simulink model "sschdlexSwissRectifierModel"  (R2026a)
settings: Solver=FixedStepDiscrete  StopTime=.03  AbsTol=1e-3
PostLoadFcn:
  | SolverConfiguration1_Gs = Simulink.Parameter;
  | SolverConfiguration1_Gs.Value = 1;
  | SolverConfiguration1_s = Simulink.Parameter;
  | SolverConfiguration1_s.Value = 1;
InitFcn:
  | freqMain = 50;
  | Vrms=230;
  | Vin = Vrms * sqrt(2);
  | Vout=325;
  | freqSwitch=20e3;
  | PoutMax = 7.5e3;
  | loadPercent = 50;
  | RLoad = Vout^2/(PoutMax*(loadPercent/100));
  | COut = 470e-6;
  | LDC = 305e-6;
  | LF = 85e-6;
  | CF = 4.4e-6;
undefined symbols (not defined in the file or in its folder): Down, Up
libraries: fl_lib x36, SimscapeFPGAHIL_lib x22, nesl_utility x9, simulink x2, slpidlib x2, eeGeneralControl x1
settings Model: DataTypeOverride=Off  Creator=The MathWorks, Inc.  LastModifiedBy=The MathWorks, Inc.
settings OptimizationCC: ConditionallyExecuteInputs=off
settings DebuggingCC: AlgebraicLoopMsg=error  SingleTaskRateTransMsg=error  PregeneratedLibrarySubsystemCodeDiagnostic=none
settings HardwareCC: ProdHWDeviceType=ASIC/FPGA->ASIC/FPGA  TargetBitPerLong=64.0  TargetBitPerPointer=64.0  TargetBitPerSizeT=64.0  TargetBitPerPtrDiffT=64.0  TargetLongLongMode=on  TargetIntDivRoundTo=Zero  TargetEndianess=LittleEndian  TargetWordSize=64.0  TargetHWDeviceType=Custom Processor->MATLAB Host Computer  ProdEqTarget=off
settings SimscapeCC: SimscapeNominalValues="[{\"value\":\"1\",\"unit\":\"A\"},{\"value\":\"1\",\"unit\":\"bar\"},{\"value\":\"1\",\"unit\":\"cm^2\"},{\"value\":\"1\",\"unit\":\"cm^3/s\"},{\"value\":\"1\",\"unit\":\"kJ/kg\"},{\"value\":\"1\",\"unit\":\"kW\"},{\"value\":\"1\",\"unit\":\"l\"},{\"value\":\"1\",\"unit\":\"N\"},{\"value\":\"1\",\"unit\":\"N*m\"},{\"value\":\"1\",\"unit\":\"V\"}]"

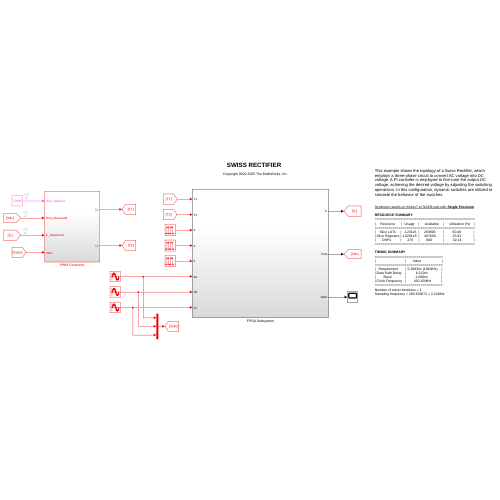
[thumbnail: Simulink's stored preview of the top-level diagram]
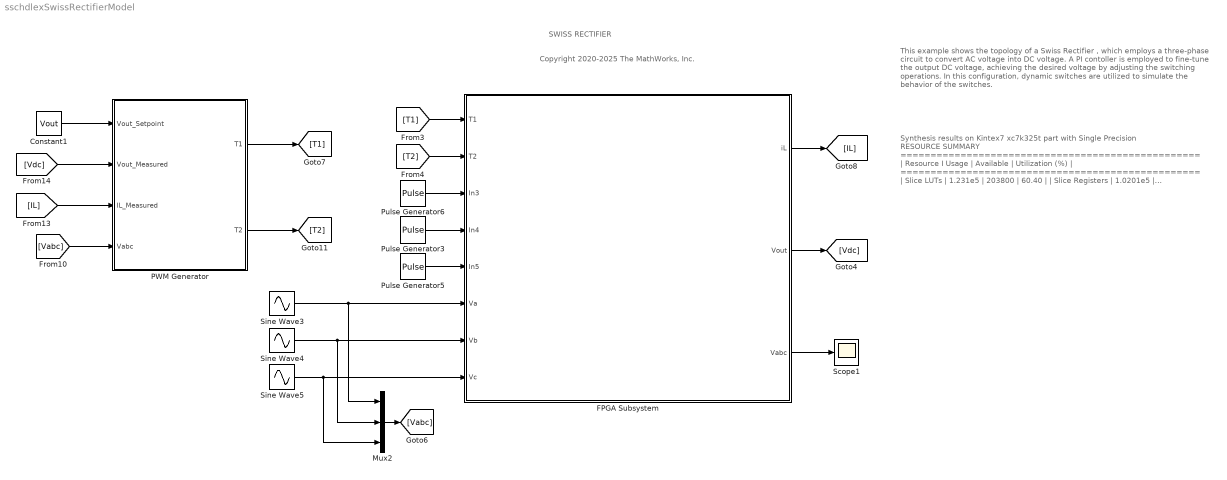
== system sschdlexSwissRectifierModel ==
  note: SWISS RECTIFIER
  note: This example shows the topology of a Swiss Rectifier , which employs a three-phase circuit to convert AC voltage into DC voltage. A PI contoller is employed to fine-tune the output DC voltage, achieving the desired voltage by adjusting the switching operations. In this configuration, dynamic switches are utilized to simulate the behavior of the switches.
  note: Copyright 2020-2025 The MathWorks, Inc.
  note: Synthesis results on Kintex7 xc7k325t part with Single Precision
      |
      | RESOURCE SUMMARY
      | ==================================================
      | | Resource I Usage | Available | Utilization (%) |
      | ==================================================
      | | Slice LUTs | 1.231e5 | 203800 | 60.40 |
      | | Slice Registers | 1.0201e5 | 407600 | 25.03 |
      | | DSPs | 270 | 840 | 32.14 |
      | ==================================================
      |
      | TIMING SUMMARY
      | ==================================
      | | | Value |
      | ==================================
      | | Requirement | 5.2083ns (192MHz) |
      | | Data Path Delay | 6.212ns |
      | | Slack | -1.036ns |
      | | Clock Frequency | 160.15MHz |
      | ==================================
      | Number of solver iterations = 1
      | Sampling frequency = 160.15M/72 = 2.22MHz
  Constant1 : Constant  Value=Vout  SampleTime=-1
  FPGA Subsystem : Subsystem
  Mux2 : Mux  Inputs=3
  PWM Generator : Subsystem
  Pulse Generator3 : DiscretePulseGenerator  Period=freqSwitch*100/(2*freqMain)  PulseWidth=round(freqSwitch*100/(2*freqMain)/3)  PhaseDelay=freqSwitch*100*(2/3-1/6)*1/(2*freqMain)  SampleTime=1/freqSwitch/100
  Pulse Generator5 : DiscretePulseGenerator  Period=freqSwitch*100/(2*freqMain)  PulseWidth=round(freqSwitch*100/(2*freqMain)/3)  PhaseDelay=round((1/3-1/6)*1/(2*freqMain)*freqSwitch*100)  SampleTime=1/freqSwitch/100
  Pulse Generator6 : DiscretePulseGenerator  Period=freqSwitch*100/(2*freqMain)  PulseWidth=round(freqSwitch*100/(2*freqMain)/3)  PhaseDelay=round(freqSwitch*100*(0/3-1/6)*1/(2*freqMain))  SampleTime=1/freqSwitch/100
  Scope1 : Scope
      settings: ActiveDisplayYMinimum=-406.58639918330113  ActiveDisplayYMaximum=406.58639918311314
  Sine Wave3 : Sin  Amplitude=Vin  Frequency=freqMain*2*pi  SampleTime=1/freqSwitch/100
  Sine Wave4 : Sin  Amplitude=Vin  Frequency=freqMain*2*pi  Phase=-120*pi/180  SampleTime=1/freqSwitch/100
  Sine Wave5 : Sin  Amplitude=Vin  Frequency=freqMain*2*pi  Phase=120*pi/180  SampleTime=1/freqSwitch/100
  wires:
  PWM Generator/1(T1) -> [T1]
  Sine Wave5/1 -> FPGA Subsystem/8(Vc), Mux2/3
  Sine Wave3/1 -> FPGA Subsystem/6(Va), Mux2/1
  [Vabc] -> PWM Generator/4(Vabc)
  Sine Wave4/1 -> Mux2/2, FPGA Subsystem/7(Vb)
  PWM Generator/2(T2) -> [T2]
  [IL] -> PWM Generator/3(IL_Measured)
  Constant1/1 -> PWM Generator/1(Vout_Setpoint)
  Mux2/1 -> [Vabc]
  [Vdc] -> PWM Generator/2(Vout_Measured)
  [T1] -> FPGA Subsystem/1(T1)
  [T2] -> FPGA Subsystem/2(T2)
  FPGA Subsystem/1(iL) -> [IL]
  FPGA Subsystem/2(Vout) -> [Vdc]
  FPGA Subsystem/3(Vabc) -> Scope1/1
  Pulse Generator3/1 -> FPGA Subsystem/4(In4)
  Pulse Generator5/1 -> FPGA Subsystem/5(In5)
  Pulse Generator6/1 -> FPGA Subsystem/3(In3)

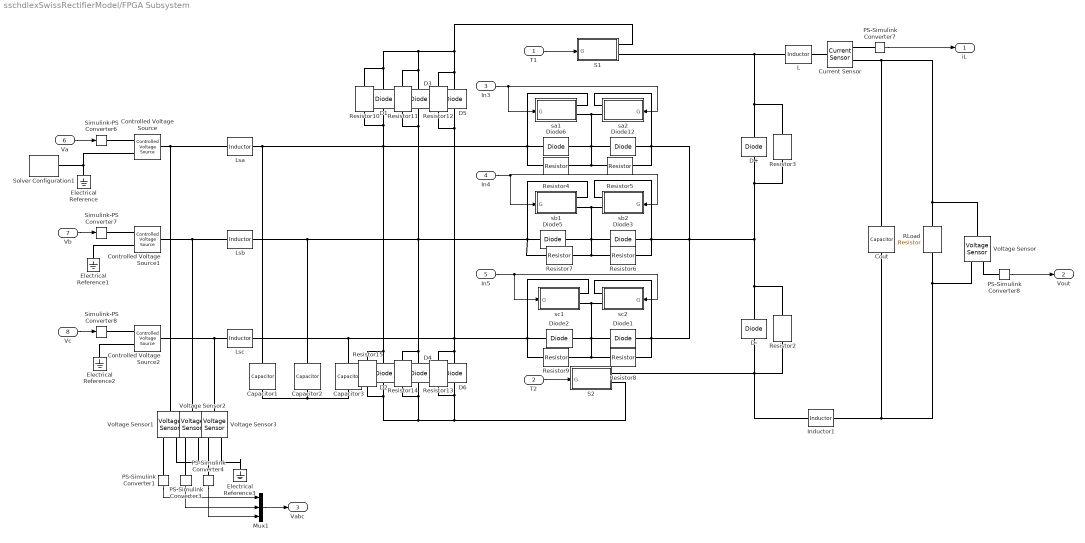
== system sschdlexSwissRectifierModel/FPGA Subsystem ==
  T1 : Inport
  T2 : Inport  Port=2
  In3 : Inport  Port=3
  In4 : Inport  Port=4
  In5 : Inport  Port=5
  Va : Inport  Port=6
  Vb : Inport  Port=7
  Vc : Inport  Port=8
  Capacitor1 : fl_lib/Electrical/Electrical Elements/Capacitor  c=CF F  r=1e-6 Ohm  g=0 1/Ohm  i_specify=off  i_priority=None  i=0 A  i_nominal_specify=off  i_nominal_value=1  i_nominal_unit=A  v_specify=off  v_priority=None  v=0 V  v_nominal_specify=off  v_nominal_value=1  v_nominal_unit=V  vc_specify=off  vc_priority=High  vc=0 V  vc_nominal_specify=off  vc_nominal_value=1  vc_nominal_unit=V
  Capacitor2 : fl_lib/Electrical/Electrical Elements/Capacitor  c=CF F  r=1e-6 Ohm  g=0 1/Ohm  i_specify=off  i_priority=None  i=0 A  i_nominal_specify=off  i_nominal_value=1  i_nominal_unit=A  v_specify=off  v_priority=None  v=0 V  v_nominal_specify=off  v_nominal_value=1  v_nominal_unit=V  vc_specify=off  vc_priority=High  vc=0 V  vc_nominal_specify=off  vc_nominal_value=1  vc_nominal_unit=V
  Capacitor3 : fl_lib/Electrical/Electrical Elements/Capacitor  c=CF F  r=1e-6 Ohm  g=0 1/Ohm  i_specify=off  i_priority=None  i=0 A  i_nominal_specify=off  i_nominal_value=1  i_nominal_unit=A  v_specify=off  v_priority=None  v=0 V  v_nominal_specify=off  v_nominal_value=1  v_nominal_unit=V  vc_specify=off  vc_priority=High  vc=0 V  vc_nominal_specify=off  vc_nominal_value=1  vc_nominal_unit=V
  Controlled Voltage Source : fl_lib/Electrical/Electrical Sources/Controlled Voltage Source
  Controlled Voltage Source1 : fl_lib/Electrical/Electrical Sources/Controlled Voltage Source
  Controlled Voltage Source2 : fl_lib/Electrical/Electrical Sources/Controlled Voltage Source
  Cout : fl_lib/Electrical/Electrical Elements/Capacitor  c=COut F  r=1e-6 Ohm  g=0 1/Ohm  i_specify=off  i_priority=None  i=0 A  i_nominal_specify=off  i_nominal_value=1  i_nominal_unit=A  v_specify=off  v_priority=None  v=0 V  v_nominal_specify=off  v_nominal_value=1  v_nominal_unit=V  vc_specify=off  vc_priority=High  vc=400 V  vc_nominal_specify=off  vc_nominal_value=1  vc_nominal_unit=V
  Current Sensor : fl_lib/Electrical/Electrical Sensors/Current Sensor
  D+ : SimscapeFPGAHIL_lib/Dynamic Switch Models/Diode  Vf=0.8  Gs=SolverConfiguration1_Gs  s=SolverConfiguration1_s
  D- : SimscapeFPGAHIL_lib/Dynamic Switch Models/Diode  Vf=0.8  Gs=SolverConfiguration1_Gs  s=SolverConfiguration1_s
  D{1..6} (6 alike) : SimscapeFPGAHIL_lib/Dynamic Switch Models/Diode  Vf=0.8  Gs=SolverConfiguration1_Gs  s=SolverConfiguration1_s
  Diode{1..3,5..6,12} (6 alike) : SimscapeFPGAHIL_lib/Dynamic Switch Models/Diode  Vf=0.8  Gs=SolverConfiguration1_Gs  s=SolverConfiguration1_s
  Electrical Reference{,1..3} (4 alike) : fl_lib/Electrical/Electrical Elements/Electrical Reference
  Inductor1 : fl_lib/Electrical/Electrical Elements/Inductor  l=LDC H  r=0 Ohm  g=1e-9 1/Ohm  i_specify=off  i_priority=None  i=0 A  i_nominal_specify=off  i_nominal_value=1  i_nominal_unit=A  v_specify=off  v_priority=None  v=0 V  v_nominal_specify=off  v_nominal_value=1  v_nominal_unit=V  i_L_specify=off  i_L_priority=High  i_L=0 A  i_L_nominal_specify=off  i_L_nominal_value=1  i_L_nominal_unit=A
  L : fl_lib/Electrical/Electrical Elements/Inductor  l=LDC H  r=0 Ohm  g=1e-9 1/Ohm  i_specify=off  i_priority=None  i=0 A  i_nominal_specify=off  i_nominal_value=1  i_nominal_unit=A  v_specify=off  v_priority=None  v=0 V  v_nominal_specify=off  v_nominal_value=1  v_nominal_unit=V  i_L_specify=off  i_L_priority=High  i_L=0 A  i_L_nominal_specify=off  i_L_nominal_value=1  i_L_nominal_unit=A
  Lsa : fl_lib/Electrical/Electrical Elements/Inductor  l=LF H  r=0 Ohm  g=1e-9 1/Ohm  i_specify=off  i_priority=None  i=0 A  i_nominal_specify=off  i_nominal_value=1  i_nominal_unit=A  v_specify=off  v_priority=None  v=0 V  v_nominal_specify=off  v_nominal_value=1  v_nominal_unit=V  i_L_specify=off  i_L_priority=High  i_L=0 A  i_L_nominal_specify=off  i_L_nominal_value=1  i_L_nominal_unit=A
  Lsb : fl_lib/Electrical/Electrical Elements/Inductor  l=LF H  r=0 Ohm  g=1e-9 1/Ohm  i_specify=off  i_priority=None  i=0 A  i_nominal_specify=off  i_nominal_value=1  i_nominal_unit=A  v_specify=off  v_priority=None  v=0 V  v_nominal_specify=off  v_nominal_value=1  v_nominal_unit=V  i_L_specify=off  i_L_priority=High  i_L=0 A  i_L_nominal_specify=off  i_L_nominal_value=1  i_L_nominal_unit=A
  Lsc : fl_lib/Electrical/Electrical Elements/Inductor  l=LF H  r=0 Ohm  g=1e-9 1/Ohm  i_specify=off  i_priority=None  i=0 A  i_nominal_specify=off  i_nominal_value=1  i_nominal_unit=A  v_specify=off  v_priority=None  v=0 V  v_nominal_specify=off  v_nominal_value=1  v_nominal_unit=V  i_L_specify=off  i_L_priority=High  i_L=0 A  i_L_nominal_specify=off  i_L_nominal_value=1  i_L_nominal_unit=A
  Mux1 : Mux  Inputs=3
  PS-Simulink Converter{1,3..4,7..8} (5 alike) : nesl_utility/PS-Simulink Converter  PhysicalDomain=network_engine_domain  SubClassName=ps_output  LeftPortType=input  RightPortType=output  PseudoPeriodic=off  Frequencies=[]  VectorFormat=1-D array  Unit=1  AffineConversion=off
  RLoad : fl_lib/Electrical/Electrical Elements/Resistor  R=RLoad Ohm  i_specify=off  i_priority=None  i=0 A  i_nominal_specify=off  i_nominal_value=1  i_nominal_unit=A  v_specify=off  v_priority=None  v=0 V  v_nominal_specify=off  v_nominal_value=1  v_nominal_unit=V
  Resistor{2..15} (14 alike) : fl_lib/Electrical/Electrical Elements/Resistor  R=500 Ohm  i_specify=off  i_priority=None  i=0 A  i_nominal_specify=off  i_nominal_value=1  i_nominal_unit=A  v_specify=off  v_priority=None  v=0 V  v_nominal_specify=off  v_nominal_value=1  v_nominal_unit=V
  S1 : Subsystem
  S2 : Subsystem
  Simulink-PS Converter6 : nesl_utility/Simulink-PS Converter  PhysicalDomain=network_engine_domain  SubClassName=ps_input  LeftPortType=input  RightPortType=output  PseudoPeriodic=off  Frequencies=[]  NoiseDistribution=none  NoiseParameters=[]  Unit=1  AffineConversion=off  FilteringAndDerivatives=provide  SimscapeFilterOrder=1  InputFilterTimeConstant=0.001  UdotUserProvided=0
  Simulink-PS Converter7 : nesl_utility/Simulink-PS Converter  PhysicalDomain=network_engine_domain  SubClassName=ps_input  LeftPortType=input  RightPortType=output  PseudoPeriodic=off  Frequencies=[]  NoiseDistribution=none  NoiseParameters=[]  Unit=1  AffineConversion=off  FilteringAndDerivatives=provide  SimscapeFilterOrder=1  InputFilterTimeConstant=0.001  UdotUserProvided=0
  Simulink-PS Converter8 : nesl_utility/Simulink-PS Converter  PhysicalDomain=network_engine_domain  SubClassName=ps_input  LeftPortType=input  RightPortType=output  PseudoPeriodic=off  Frequencies=[]  NoiseDistribution=none  NoiseParameters=[]  Unit=1  AffineConversion=off  FilteringAndDerivatives=provide  SimscapeFilterOrder=1  InputFilterTimeConstant=0.001  UdotUserProvided=0
  Solver Configuration1 : nesl_utility/Solver Configuration  PhysicalDomain=network_engine_domain  SubClassName=solver  LeftPortType=input  RightPortType=generic  Tones=[]  Harmonics=[]  SimulateNoise=off  Profile=off  UseLocalSampling=off  EnableSwitchedLinearOptims=on  FrequencyDomain=off  UseCCode=off  RelTol=0.001  AbsTol=1e-06  MinStep=1e-09  ToWorkspace=off  RevertToSquareIcSolve=off  NumHomotopyIterations=100  PhasorMode=off  PhasorModeNumHarmonics=1  ConsistencySolver=NEWTON_FTOL  CanonicalOrdering=UNORDERED  OptimizeIntermediates=UNOPTIMIZED  IndexReductionMethod=DerivativeReplacement  DoDC=off  ResidualTolerance=1e-09  ConsistencyTolSource=GLOBAL  ConsistencyAbsTol=0.001  ConsistencyRelTol=0.001  ConsistencyTolFactor=0.001  UseLocalSolver=on  LocalSolverChoice=NE_BACKWARD_EULER_ADVANCER  ResolveIndetEquations=on  FunctionEvalNumThread=1  LocalSolverSampleTime=1/freqSwitch/100  DoFixedCost=off  MaxNonlinIter=3  MaxModeIter=2  ComputeImpulses=off  ImpulseIterations=2  LinearAlgebra=auto  LinearAlgebraNumThread=0  EquationFormulation=NE_TIME_EF  DelaysMemoryBudget=1024  AutomaticFiltering=off  FilteringTimeConstant=0.001  PartitionStorageMethod=AS_NEEDED  PartitionMemoryBudget=1024  PartitionMethod=FAST  MultibodyUseLocalSolver=off  MultibodyLocalSolverChoice=ODE1  MultibodyLocalSolverSampleTime=0.001
  Voltage Sensor{,1..3} (4 alike) : fl_lib/Electrical/Electrical Sensors/Voltage Sensor
  sa1 : Subsystem
  sa2 : Subsystem
  sb1 : Subsystem
  sb2 : Subsystem
  sc1 : Subsystem
  sc2 : Subsystem
  iL : Outport
  Vout : Outport  Port=2
  Vabc : Outport  Port=3
  wires:
  In3/1 -> sa1/1(G), sa2/1(G)
  In4/1 -> sb1/1(G), sb2/1(G)
  PS-Simulink Converter8/1 -> Vout/1
  In5/1 -> sc2/1(G), sc1/1(G)
  T1/1 -> S1/1(G)
  Vc/1 -> Simulink-PS Converter8/1
  Vb/1 -> Simulink-PS Converter7/1
  T2/1 -> S2/1(G)
  Va/1 -> Simulink-PS Converter6/1
  PS-Simulink Converter7/1 -> iL/1
  PS-Simulink Converter1/1 -> Mux1/1
  PS-Simulink Converter3/1 -> Mux1/2
  PS-Simulink Converter4/1 -> Mux1/3
  Mux1/1 -> Vabc/1
  connections:
  Simulink-PS Converter8/RConn1 -- Controlled Voltage Source2/RConn1
  Capacitor3/RConn1 -- Capacitor1/RConn1 -- Capacitor2/RConn1
  Resistor3/LConn1 -- D+/RConn1 -- L/LConn1 -- S1/RConn2
  Resistor6/RConn1 -- Resistor7/LConn1 -- sb2/RConn2 -- sb1/RConn2 -- Diode5/LConn1 -- Diode3/LConn1
  Resistor10/RConn1 -- D1/RConn1 -- Resistor11/RConn1 -- D3/RConn1 -- Resistor12/RConn1 -- D5/RConn1 -- S1/RConn1
  Resistor12/LConn1 -- D5/LConn1 -- Resistor9/RConn1 -- Diode2/RConn1 -- sc1/RConn1 -- Lsc/RConn1 -- Capacitor3/LConn1 -- Resistor13/RConn1 -- D6/RConn1
  Resistor15/LConn1 -- D2/LConn1 -- Resistor14/LConn1 -- D4/LConn1 -- Resistor13/LConn1 -- D6/LConn1 -- S2/RConn2
  Voltage Sensor2/LConn1 -- Lsb/LConn1 -- Controlled Voltage Source1/LConn1
  Resistor3/RConn1 -- D+/LConn1 -- Resistor2/LConn1 -- D-/RConn1 -- Diode12/RConn1 -- sa2/RConn1 -- Resistor5/LConn1 -- Resistor8/LConn1 -- sc2/RConn1 -- Diode1/RConn1 -- Diode3/RConn1 -- sb2/RConn1 -- Resistor6/LConn1
  Voltage Sensor1/LConn1 -- Lsa/LConn1 -- Controlled Voltage Source/LConn1
  Resistor9/LConn1 -- Resistor8/RConn1 -- sc2/RConn2 -- sc1/RConn2 -- Diode1/LConn1 -- Diode2/LConn1
  RLoad/RConn1 -- Cout/RConn1 -- Inductor1/RConn1 -- Voltage Sensor/RConn2
  Resistor5/RConn1 -- Resistor4/LConn1 -- Diode6/LConn1 -- Diode12/LConn1 -- sa2/RConn2 -- sa1/RConn2
  Electrical Reference1/LConn1 -- Controlled Voltage Source1/RConn2
  L/RConn1 -- Current Sensor/LConn1
  Simulink-PS Converter6/RConn1 -- Controlled Voltage Source/RConn1
  Resistor10/LConn1 -- D1/LConn1 -- Resistor15/RConn1 -- D2/RConn1 -- Lsa/RConn1 -- Capacitor1/LConn1 -- sa1/RConn1 -- Resistor4/RConn1 -- Diode6/RConn1
  Voltage Sensor3/LConn1 -- Lsc/LConn1 -- Controlled Voltage Source2/LConn1
  Solver Configuration1/RConn1 -- Controlled Voltage Source/RConn2 -- Electrical Reference/LConn1
  Resistor7/RConn1 -- Diode5/RConn1 -- sb1/RConn1 -- Resistor11/LConn1 -- D3/LConn1 -- Capacitor2/LConn1 -- Lsb/RConn1 -- Resistor14/RConn1 -- D4/RConn1
  PS-Simulink Converter7/LConn1 -- Current Sensor/RConn1
  PS-Simulink Converter8/LConn1 -- Voltage Sensor/RConn1
  Inductor1/LConn1 -- Resistor2/RConn1 -- D-/LConn1 -- S2/RConn1
  Electrical Reference2/LConn1 -- Controlled Voltage Source2/RConn2
  Cout/LConn1 -- Current Sensor/RConn2 -- RLoad/LConn1 -- Voltage Sensor/LConn1
  Simulink-PS Converter7/RConn1 -- Controlled Voltage Source1/RConn1
  Voltage Sensor2/RConn2 -- Electrical Reference3/LConn1 -- Voltage Sensor3/RConn2 -- Voltage Sensor1/RConn2
  PS-Simulink Converter1/LConn1 -- Voltage Sensor1/RConn1
  PS-Simulink Converter4/LConn1 -- Voltage Sensor3/RConn1
  PS-Simulink Converter3/LConn1 -- Voltage Sensor2/RConn1

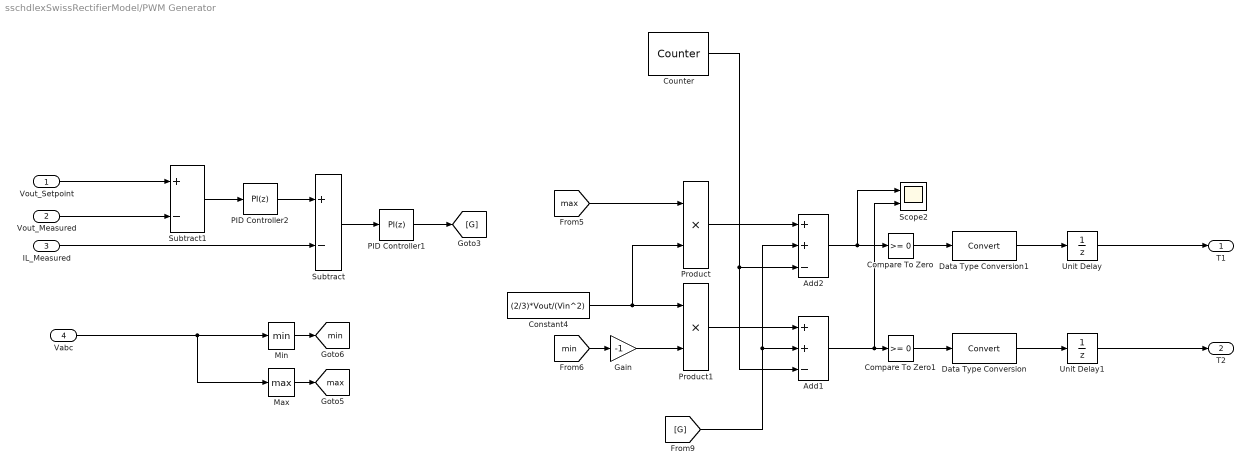
== system sschdlexSwissRectifierModel/PWM Generator ==
  Vout_Setpoint : Inport
  Vout_Measured : Inport  Port=2
  IL_Measured : Inport  Port=3
  Vabc : Inport  Port=4
  Add1 : Sum  Inputs=++-
  Add2 : Sum  Inputs=++-
  Compare To Zero : simulink/Logic and Bit Operations/Compare To Zero  relop=>=  OutDataTypeStr=boolean
  Compare To Zero1 : simulink/Logic and Bit Operations/Compare To Zero  relop=>=  OutDataTypeStr=boolean
  Constant4 : Constant  Value=(2/3)*Vout/(Vin^2)  SampleTime=-1
  Counter : eeGeneralControl/Counter  CarrCount=Up-Down  Range=[-1 1]  Tper=1/(2*freqSwitch)  Tdelay=0  Ts=1/freqSwitch/100
      settings: LibrarySourceBlock=ee_sl_lib/General Control/Counter
  Data Type Conversion : DataTypeConversion  SaturateOnIntegerOverflow=off  RndMeth=Floor
  Data Type Conversion1 : DataTypeConversion  SaturateOnIntegerOverflow=off  RndMeth=Floor
  Gain : Gain  Gain=-1
  Max : MinMax  Function=max
  Min : MinMax
  PID Controller1 : slpidlib/PID Controller  Controller=PI  Form=Parallel  TimeDomain=Discrete-time  UseExternalTs=off  SampleTime=-1  IntegratorMethod=Forward Euler  FilterMethod=Forward Euler  ControllerParametersSource=internal  P=0.1  I=10000/5  UseKiTs=off  D=0  UseExternalDerivativeSource=off  N=100  UseFilter=on  TunerSelectOption=Transfer Function Based (PID Tuner App)  InitialConditionSource=internal  InitialConditionForIntegrator=0  InitialConditionForFilter=0  DifferentiatorICPrevScaledInput=0  ExternalReset=none  TrackingMode=off  Kt=1  LimitOutput=off  SatLimitsSource=internal  UpperSaturationLimit=inf  LowerSaturationLimit=-inf  LinearizeAsGain=on  AntiWindupMode=none  Kb=1  LimitIntegrator=off  UpperIntegratorSaturationLimit=inf  LowerIntegratorSaturationLimit=-inf  POutMin=[]  POutMax=[]  IOutMin=[]  IOutMax=[]  DOutMin=[]  DOutMax=[]  NOutMin=[]  NOutMax=[]  SumOutMin=[]  SumOutMax=[]  SaturationOutMin=[]  SaturationOutMax=[]  PParamMin=[]  PParamMax=[]  IParamMin=[]  IParamMax=[]  DParamMin=[]  DParamMax=[]  NParamMin=[]  NParamMax=[]  KbParamMin=[]  KbParamMax=[]  KtParamMin=[]  KtParamMax=[]  KbOutMin=[]  KbOutMax=[]  KtOutMin=[]  KtOutMax=[]  IntegratorOutMin=[]  IntegratorOutMax=[]  FilterOutMin=[]  FilterOutMax=[]  SumI1OutMin=[]  SumI1OutMax=[]  SumI2OutMin=[]  SumI2OutMax=[]  SumI3OutMin=[]  SumI3OutMax=[]  SumI4OutMin=[]  SumI4OutMax=[]  SumDOutMin=[]  SumDOutMax=[]  DifferentiatorOutMin=[]  DifferentiatorOutMax=[]  FilterDiffOutCoefMin=[]  FilterDiffOutCoefMax=[]  ReciprocalOutMin=[]  ReciprocalOutMax=[]  SumDenOutMin=[]  SumDenOutMax=[]  SumNumOutMin=[]  SumNumOutMax=[]  DivideOutMin=[]  DivideOutMax=[]  UdiffTsProdOutMin=[]  UdiffTsProdOutMax=[]  NTsProdOutMin=[]  NTsProdOutMax=[]  UintegralTsProdOutMin=[]  UintegralTsProdOutMax=[]  UngainTsProdOutMin=[]  UngainTsProdOutMax=[]  ClampingZeroOutDataTypeStr=Inherit: Inherit via back propagation  ClampingZeroOutMin=[]  ClampingZeroOutMax=[]  FilterDenConstantOutDataTypeStr=Inherit: Inherit via back propagation  FilterDenConstantOutMin=[]  FilterDenConstantOutMax=[]  PCopyOutDataTypeStr=Inherit: Inherit via back propagation  PCopyOutMin=[]  PCopyOutMax=[]  NCopyOutDataTypeStr=Inherit: Inherit via back propagation  NCopyOutMin=[]  NCopyOutMax=[]  IntegratorContinuousStateAttributes=''  IntegratorStateMustResolveToSignalObject=off  IntegratorRTWStateStorageClass=Auto  FilterContinuousStateAttributes=''  FilterStateMustResolveToSignalObject=off  FilterRTWStateStorageClass=Auto  ParallelPVariant=InternalParameters  IdealPVariant=Disabled  IVariant=InternalParameters  DVariant=Disabled  IntegratorVariant=Discrete  SatVariant=Disabled  AWVariant=Passthrough  PCopyVariant=Disabled  TRVariant=Disabled  FdbkBlocksVariant=Forward  IdealPFdbkVariant=Disabled  SatFdbkVariant=Disabled  DerivativeFilterVariant=Disabled  NVariant=Disabled  NCopyVariant=Disabled_SignalSpec  FilterICVariant=Disabled  IntegratorICVariant=InternalICs  ExternalResetVariant=Disabled  TRSumVariant=Passthrough  SumFdbkVariant=Disabled  SumVariant=Sum_PI  TsampFilterVariant=InternalTs  TsampNgainVariant=Passthrough  TsampIntegralVariant=Disabled_SignalSpec  ExternalSaturationOutDataTypeStr=Inherit: Same as second input  DerivativeSourceVariant=Disabled  PreIntVariant=InternalPreInt
  PID Controller2 : slpidlib/PID Controller  Controller=PI  Form=Parallel  TimeDomain=Discrete-time  UseExternalTs=off  SampleTime=-1  IntegratorMethod=Forward Euler  FilterMethod=Forward Euler  ControllerParametersSource=internal  P=1/10  I=10  UseKiTs=off  D=0  UseExternalDerivativeSource=off  N=100  UseFilter=on  TunerSelectOption=Transfer Function Based (PID Tuner App)  InitialConditionSource=internal  InitialConditionForIntegrator=0  InitialConditionForFilter=0  DifferentiatorICPrevScaledInput=0  ExternalReset=none  TrackingMode=off  Kt=1  LimitOutput=off  SatLimitsSource=internal  UpperSaturationLimit=inf  LowerSaturationLimit=-inf  LinearizeAsGain=on  AntiWindupMode=none  Kb=1  LimitIntegrator=off  UpperIntegratorSaturationLimit=inf  LowerIntegratorSaturationLimit=-inf  POutMin=[]  POutMax=[]  IOutMin=[]  IOutMax=[]  DOutMin=[]  DOutMax=[]  NOutMin=[]  NOutMax=[]  SumOutMin=[]  SumOutMax=[]  SaturationOutMin=[]  SaturationOutMax=[]  PParamMin=[]  PParamMax=[]  IParamMin=[]  IParamMax=[]  DParamMin=[]  DParamMax=[]  NParamMin=[]  NParamMax=[]  KbParamMin=[]  KbParamMax=[]  KtParamMin=[]  KtParamMax=[]  KbOutMin=[]  KbOutMax=[]  KtOutMin=[]  KtOutMax=[]  IntegratorOutMin=[]  IntegratorOutMax=[]  FilterOutMin=[]  FilterOutMax=[]  SumI1OutMin=[]  SumI1OutMax=[]  SumI2OutMin=[]  SumI2OutMax=[]  SumI3OutMin=[]  SumI3OutMax=[]  SumI4OutMin=[]  SumI4OutMax=[]  SumDOutMin=[]  SumDOutMax=[]  DifferentiatorOutMin=[]  DifferentiatorOutMax=[]  FilterDiffOutCoefMin=[]  FilterDiffOutCoefMax=[]  ReciprocalOutMin=[]  ReciprocalOutMax=[]  SumDenOutMin=[]  SumDenOutMax=[]  SumNumOutMin=[]  SumNumOutMax=[]  DivideOutMin=[]  DivideOutMax=[]  UdiffTsProdOutMin=[]  UdiffTsProdOutMax=[]  NTsProdOutMin=[]  NTsProdOutMax=[]  UintegralTsProdOutMin=[]  UintegralTsProdOutMax=[]  UngainTsProdOutMin=[]  UngainTsProdOutMax=[]  ClampingZeroOutDataTypeStr=Inherit: Inherit via back propagation  ClampingZeroOutMin=[]  ClampingZeroOutMax=[]  FilterDenConstantOutDataTypeStr=Inherit: Inherit via back propagation  FilterDenConstantOutMin=[]  FilterDenConstantOutMax=[]  PCopyOutDataTypeStr=Inherit: Inherit via back propagation  PCopyOutMin=[]  PCopyOutMax=[]  NCopyOutDataTypeStr=Inherit: Inherit via back propagation  NCopyOutMin=[]  NCopyOutMax=[]  IntegratorContinuousStateAttributes=''  IntegratorStateMustResolveToSignalObject=off  IntegratorRTWStateStorageClass=Auto  FilterContinuousStateAttributes=''  FilterStateMustResolveToSignalObject=off  FilterRTWStateStorageClass=Auto  ParallelPVariant=InternalParameters  IdealPVariant=Disabled  IVariant=InternalParameters  DVariant=Disabled  IntegratorVariant=Discrete  SatVariant=Disabled  AWVariant=Passthrough  PCopyVariant=Disabled  TRVariant=Disabled  FdbkBlocksVariant=Forward  IdealPFdbkVariant=Disabled  SatFdbkVariant=Disabled  DerivativeFilterVariant=Disabled  NVariant=Disabled  NCopyVariant=Disabled_SignalSpec  FilterICVariant=Disabled  IntegratorICVariant=InternalICs  ExternalResetVariant=Disabled  TRSumVariant=Passthrough  SumFdbkVariant=Disabled  SumVariant=Sum_PI  TsampFilterVariant=InternalTs  TsampNgainVariant=Passthrough  TsampIntegralVariant=Disabled_SignalSpec  ExternalSaturationOutDataTypeStr=Inherit: Same as second input  DerivativeSourceVariant=Disabled  PreIntVariant=InternalPreInt
  Product : Product
  Product1 : Product
  Scope2 : Scope  NumInputPorts=2
      settings: ActiveDisplayYMinimum=-1.63789  ActiveDisplayYMaximum=2.02198  DataLoggingVariableName=ScopeData4
  Subtract : Sum  Inputs=+-
  Subtract1 : Sum  Inputs=+-
  Unit Delay : UnitDelay  SampleTime=-1
  Unit Delay1 : UnitDelay  SampleTime=-1
  T1 : Outport  VectorParamsAs1DForOutWhenUnconnected=off
  T2 : Outport  Port=2  VectorParamsAs1DForOutWhenUnconnected=off
  tag scope: max=global, min=global
  wires:
  Vabc/1 -> Max/1, Min/1
  Constant4/1 -> Product/2, Product1/1
  Compare To Zero1/1 -> Data Type Conversion/1
  [G] -> Add2/2, Add1/2
  Unit Delay1/1 -> T2/1
  IL_Measured/1 -> Subtract/2
  PID Controller2/1 -> Subtract/1
  Compare To Zero/1 -> Data Type Conversion1/1
  Add1/1 -> Compare To Zero1/1, Scope2/2
  Add2/1 -> Compare To Zero/1, Scope2/1
  Product/1 -> Add2/1
  Data Type Conversion1/1 -> Unit Delay/1
  Counter/1 -> Add2/3, Add1/3
  [max] -> Product/1
  Subtract/1 -> PID Controller1/1
  Product1/1 -> Add1/1
  Data Type Conversion/1 -> Unit Delay1/1
  Gain/1 -> Product1/2
  Max/1 -> [max]
  Min/1 -> [min]
  Subtract1/1 -> PID Controller2/1
  [min] -> Gain/1
  PID Controller1/1 -> [G]
  Vout_Measured/1 -> Subtract1/2
  Vout_Setpoint/1 -> Subtract1/1
  Unit Delay/1 -> T1/1

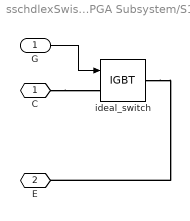
== system sschdlexSwissRectifierModel/FPGA Subsystem/S1 ==
  G : Inport
  ideal_switch : SimscapeFPGAHIL_lib/Dynamic Switch Models/IGBT  Vf=0.8  Vth=0.5  Gs=SolverConfiguration1_Gs  s=SolverConfiguration1_s
  C : PMIOPort  Side=Right
  E : PMIOPort  Port=2  Side=Right
  wires:
  G/1 -> ideal_switch/1
  connections:
  ideal_switch/RConn1 -- E/RConn1
  C/RConn1 -- ideal_switch/LConn1

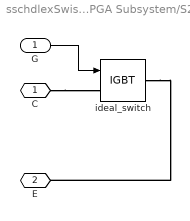
== system sschdlexSwissRectifierModel/FPGA Subsystem/S2 ==
  G : Inport
  ideal_switch : SimscapeFPGAHIL_lib/Dynamic Switch Models/IGBT  Vf=0.8  Vth=0.5  Gs=SolverConfiguration1_Gs  s=SolverConfiguration1_s
  C : PMIOPort  Side=Right
  E : PMIOPort  Port=2  Side=Right
  wires:
  G/1 -> ideal_switch/1
  connections:
  C/RConn1 -- ideal_switch/LConn1
  ideal_switch/RConn1 -- E/RConn1

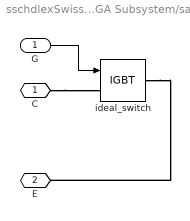
== system sschdlexSwissRectifierModel/FPGA Subsystem/sa1 ==
  G : Inport
  ideal_switch : SimscapeFPGAHIL_lib/Dynamic Switch Models/IGBT  Vf=0.8  Vth=0.5  Gs=SolverConfiguration1_Gs  s=SolverConfiguration1_s
  C : PMIOPort  Side=Right
  E : PMIOPort  Port=2  Side=Right
  wires:
  G/1 -> ideal_switch/1
  connections:
  ideal_switch/RConn1 -- E/RConn1
  C/RConn1 -- ideal_switch/LConn1

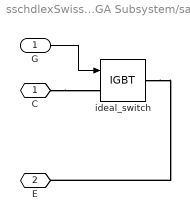
== system sschdlexSwissRectifierModel/FPGA Subsystem/sa2 ==
  G : Inport
  ideal_switch : SimscapeFPGAHIL_lib/Dynamic Switch Models/IGBT  Vf=0.8  Vth=0.5  Gs=SolverConfiguration1_Gs  s=SolverConfiguration1_s
  C : PMIOPort  Side=Right
  E : PMIOPort  Port=2  Side=Right
  wires:
  G/1 -> ideal_switch/1
  connections:
  C/RConn1 -- ideal_switch/LConn1
  ideal_switch/RConn1 -- E/RConn1

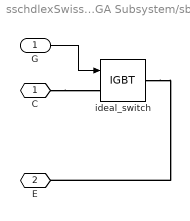
== system sschdlexSwissRectifierModel/FPGA Subsystem/sb1 ==
  G : Inport
  ideal_switch : SimscapeFPGAHIL_lib/Dynamic Switch Models/IGBT  Vf=0.8  Vth=0.5  Gs=SolverConfiguration1_Gs  s=SolverConfiguration1_s
  C : PMIOPort  Side=Right
  E : PMIOPort  Port=2  Side=Right
  wires:
  G/1 -> ideal_switch/1
  connections:
  C/RConn1 -- ideal_switch/LConn1
  ideal_switch/RConn1 -- E/RConn1

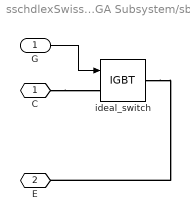
== system sschdlexSwissRectifierModel/FPGA Subsystem/sb2 ==
  G : Inport
  ideal_switch : SimscapeFPGAHIL_lib/Dynamic Switch Models/IGBT  Vf=0.8  Vth=0.5  Gs=SolverConfiguration1_Gs  s=SolverConfiguration1_s
  C : PMIOPort  Side=Right
  E : PMIOPort  Port=2  Side=Right
  wires:
  G/1 -> ideal_switch/1
  connections:
  C/RConn1 -- ideal_switch/LConn1
  ideal_switch/RConn1 -- E/RConn1

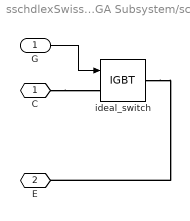
== system sschdlexSwissRectifierModel/FPGA Subsystem/sc1 ==
  G : Inport
  ideal_switch : SimscapeFPGAHIL_lib/Dynamic Switch Models/IGBT  Vf=0.8  Vth=0.5  Gs=SolverConfiguration1_Gs  s=SolverConfiguration1_s
  C : PMIOPort  Side=Right
  E : PMIOPort  Port=2  Side=Right
  wires:
  G/1 -> ideal_switch/1
  connections:
  C/RConn1 -- ideal_switch/LConn1
  ideal_switch/RConn1 -- E/RConn1

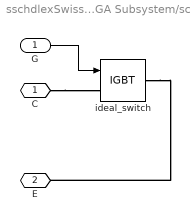
== system sschdlexSwissRectifierModel/FPGA Subsystem/sc2 ==
  G : Inport
  ideal_switch : SimscapeFPGAHIL_lib/Dynamic Switch Models/IGBT  Vf=0.8  Vth=0.5  Gs=SolverConfiguration1_Gs  s=SolverConfiguration1_s
  C : PMIOPort  Side=Right
  E : PMIOPort  Port=2  Side=Right
  wires:
  G/1 -> ideal_switch/1
  connections:
  C/RConn1 -- ideal_switch/LConn1
  ideal_switch/RConn1 -- E/RConn1
